simulink model "lin_feedback_EMPTY (1)"  (R2021b)
settings: Solver=ode1  StartTime=0.0  StopTime=tmax  FixedStep=Ts  RelTol=1e-3  EnableMultiTasking=on
values from neighbouring files (symbols this model uses):
  Kd = 0.5    [nlc_setup_solucion (1).m]    (also in nlc_setup_solucion.m = 2)
  Ki = 0    [nlc_setup_solucion (1).m]    (also in nlc_setup_solucion.m = 1)
  Kp = 1    [nlc_setup_solucion (1).m]    (also in nlc_setup_solucion.m = 2.5)
  spd_b = 0    [nlc_setup_solucion (1).m]
  spd_Kaw = spd_aw*spd_Ki/spd_Kp    (= 13.2992871582)    [nlc_setup_solucion (1).m]
  spd_Ki = wn_w^2/b_w    (= 2.87757197383)    [nlc_setup_solucion (1).m]
  spd_Kp = (2*zeta_w*wn_w - a_w)/b_w    (= 0.216370391856)    [nlc_setup_solucion (1).m]
  tau_lpf = 0    [nlc_setup_solucion (1).m]
  Ts = 0.002    [nlc_setup_solucion (1).m]    (also in nlc_setup_solucion.m)
  w_max = 380    [nlc_setup_solucion (1).m]
  w_tau = 20    [nlc_setup_solucion (1).m]    (also in nlc_setup_solucion.m = 5)
undefined symbols (not defined in the file or in its folder): DiscIntNeverNeededParam, HIL, qc_get_step_size
libraries: quarc_library x6
settings Model: SimulationMode=external  ExtModeTrigDuration=20000  Creator=MLevis  LastModifiedBy=Professorat
settings SolverCC: AlgebraicLoopSolver=TrustRegion  PositivePriorityOrder=on  AutoInsertRateTranBlk=on
settings DataIOCC: LimitDataPoints=on  SaveFormat=StructureWithTime  ReturnWorkspaceOutputs=off
settings DebuggingCC: SolverPrmCheckMsg=warning  SFUnexpectedBacktrackingDiag=warning  SFNoUnconditionalDefaultTransitionDiag=warning  SFExecutionAtInitializationDiag=none  SFMachineParentedDataDiag=warning  ArithmeticOperatorsInVariantConditions=warning
settings ModelReferenceCC: PropagateSignalLabelsOutOfModel=off
settings SFSimCC: SimUseLocalCustomCode=off  CustomCodeUndefinedFunction=UseInterfaceOnly
settings RTWCC: Description=QUARC Win64 Target Using Toolchain  SystemTargetFile=quarc_win64.tlc  TemplateMakefile=quarc_default_tmf  RTWUseLocalCustomCode=off  Toolchain=QUARC win64 | nmake (64-bit Windows)  BuildConfiguration=Faster Runs
settings CodeAppCC: StateflowObjectComments=on
settings STFCustomTargetCC: ConcurrentExecutionCompliant=on  UseToolchainInfoCompliant=on  SystemTargetFile=quarc_win64.tlc
settings GRTTargetCC: TargetLangStandard=C89/C90 (ANSI)  ParMdlRefBuildCompliant=off  CompOptLevelCompliant=off  CombineOutputUpdateFcns=off  MatFileLogging=off  CPPClassGenCompliant=off  GRTInterface=on  ExtMode=on  ExtModeMexFile=quarc_comm
settings ConfigComp: CovMetricSettings=dw  CovSaveCumulativeToWorkspaceVar=on  CovSaveSingleToWorkspaceVar=on  CovExternalEMLEnable=off  CovSFcnEnable=off

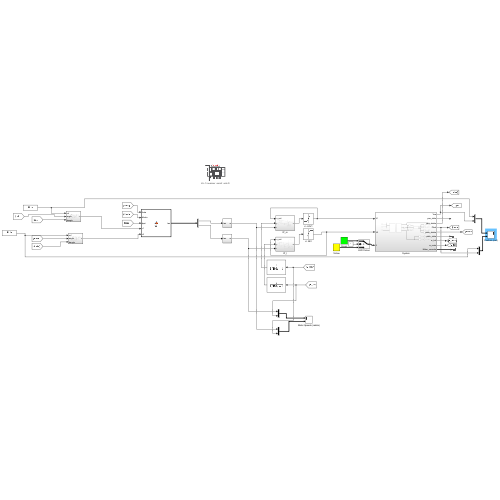
[thumbnail: Simulink's stored preview of the top-level diagram]
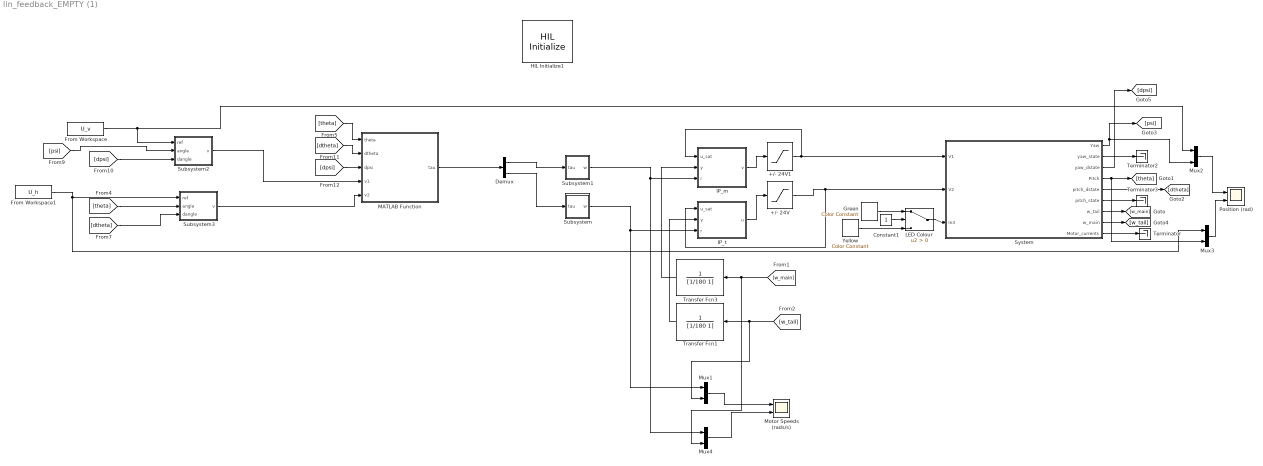
== system lin_feedback_EMPTY (1) ==
  +/- 24V : Saturate  UpperLimit=24  LowerLimit=-24
  +/- 24V1 : Saturate  UpperLimit=24  LowerLimit=-24
  Constant1 : Constant
  Demux : Demux  Outputs=2
  From Workspace : FromWorkspace  VariableName=U_v  Interpolate=off  OutputAfterFinalValue=Setting to zero
  From Workspace1 : FromWorkspace  VariableName=U_h  Interpolate=off  OutputAfterFinalValue=Setting to zero
  Green : quarc_library/Sources/Signals/Color Constant  color=[0 1 0]
      settings: SourceProductName=QUARC Targets
  HIL Initialize1 : quarc_library/Data Acquisition/Generic/Configuration/HIL Initialize  Priority=-99  object_name=HIL-1  board_type=quanser_aero2_usb  board_number=0  board_options=""  exclusive=off  active=off  hardware_clocks=[0]  clock_modes=[]  initial_clock_frequencies=[]  set_clock_params_at_start=off  set_clock_params_at_switch_in=off  set_clock_frequencies_at_start=off  set_clock_frequencies_at_switch_in=off  analog_input_channels=[0:1]  analog_input_configurations=[]  analog_input_maximums=3  analog_input_minimums=-3  set_analog_input_params_at_start=off  set_analog_input_params_at_switch_in=off  analog_output_channels=[0:1]  analog_output_maximums=24  analog_output_minimums=-24  initial_analog_outputs=[0]  final_analog_outputs=[0]  watchdog_analog_outputs=[0]  set_analog_output_params_at_start=off  set_analog_output_params_at_switch_in=off  set_analog_outputs_at_start=on  set_analog_outputs_at_switch_in=off  set_analog_outputs_at_terminate=on  set_analog_outputs_at_switch_out=off  set_analog_outputs_on_watchdog=on  digital_input_channels=[]  digital_output_channels=[0:1]  digital_output_configuration=[]  initial_digital_outputs=[1]  final_digital_outputs=[0]  watchdog_digital_outputs=[0]  set_digital_output_params_at_start=off  set_digital_output_params_at_switch_in=off  set_digital_outputs_at_start=on  set_digital_outputs_at_switch_in=off  set_digital_outputs_at_terminate=on  set_digital_outputs_at_switch_out=off  set_digital_outputs_on_watchdog=on  encoder_channels=[0:3]  quadrature=[4]  encoder_filter_frequency=[]  initial_encoder_counts=[0]  set_encoder_params_at_start=off  set_encoder_params_at_switch_in=off  set_encoder_counts_at_start=on  set_encoder_counts_at_switch_in=off  pwm_channels=[]  pwm_modes=[]  pwm_frequency=[]  pwm_configuration=[]  pwm_alignment=[]  pwm_polarity=[]  pwm_leading_deadband=[]  pwm_trailing_deadband=[]  initial_pwm_outputs=[]  final_pwm_outputs=[]  watchdog_pwm_outputs=[]  set_pwm_params_at_start=off  set_pwm_params_at_switch_in=off  set_pwm_outputs_at_start=off  set_pwm_outputs_at_switch_in=off  set_pwm_outputs_at_terminate=off  set_pwm_outputs_at_switch_out=off  set_pwm_outputs_on_watchdog=off  other_output_channels=[11000:11002]  initial_other_outputs=[0 1 0]  final_other_outputs=[1 0 0]  watchdog_other_outputs=[0 0 1]  set_other_outputs_at_start=on  set_other_outputs_at_switch_in=off  set_other_outputs_at_terminate=on  set_other_outputs_at_switch_out=off  set_other_outputs_on_watchdog=on
  IP_m : Subsystem
  IP_t : Subsystem
  LED Colour : Switch  Criteria=u2 > Threshold
  MATLAB Function : MATLAB Function  TreatAsAtomicUnit=on
  Motor Speeds (rads/s) : Scope  NumInputPorts=2
  Mux{1..4} (4 alike) : Mux  Inputs=2
  Position (rad) : Scope  NumInputPorts=2
  Subsystem : Subsystem
  Subsystem1 : Subsystem
  Subsystem2 : Subsystem
  Subsystem3 : Subsystem
  System : Subsystem
  Terminator : Terminator
  Terminator2 : Terminator
  Terminator3 : Terminator
  Transfer Fcn1 : TransferFcn  Denominator=[1/180 1]
  Transfer Fcn3 : TransferFcn  Denominator=[1/180 1]
  Yellow : quarc_library/Sources/Signals/Color Constant  color=[1 1 0]
      settings: SourceProductName=QUARC Targets
  wires:
  Green/1 -> LED Colour/1
  Yellow/1 -> LED Colour/3
  Constant1/1 -> LED Colour/2
  +/- 24V/1 -> IP_t/1(u_sat), System/2(V2)
  +/- 24V1/1 -> IP_m/1(u_sat), System/1(V1)
  IP_t/1(u) -> +/- 24V/1
  Mux1/1 -> Motor Speeds (rads/s)/1
  Mux4/1 -> Motor Speeds (rads/s)/2
  LED Colour/1 -> System/3(In3)
  System/7(w_tail) -> [w_main]
  System/8(w_main) -> [w_tail]
  System/9(Motor_currents) -> Terminator/1
  System/1(Yaw) -> [psi], Mux2/2
  System/2(yaw_state) -> Terminator2/1
  System/6(pitch_state) -> Terminator3/1
  [w_main] -> Mux4/2, Transfer Fcn3/1
  [w_tail] -> Mux1/2, Transfer Fcn1/1
  Subsystem1/1(w) -> Mux4/1, IP_m/3(r)
  Subsystem/1(w) -> Mux1/1, IP_t/3(r)
  Transfer Fcn1/1 -> IP_t/2(y)
  System/4(Pitch) -> Mux3/2, [theta]
  System/5(pitch_dstate) -> [dtheta]
  System/3(yaw_dstate) -> [dpsi]
  [theta] -> Subsystem3/2(angle)
  [dtheta] -> Subsystem3/3(dangle)
  [psi] -> Subsystem2/2(angle)
  [dpsi] -> Subsystem2/3(dangle)
  From Workspace1/1 -> Mux3/1, Subsystem3/1(ref)
  From Workspace/1 -> Subsystem2/1(ref), Mux2/1
  Mux2/1 -> Position (rad)/1
  Mux3/1 -> Position (rad)/2
  Demux/1 -> Subsystem1/1(tau)
  [dtheta] -> MATLAB Function/2(dtheta)
  Subsystem3/1(v) -> MATLAB Function/5(v2)
  Demux/2 -> Subsystem/1(tau)
  [theta] -> MATLAB Function/1(theta)
  [dpsi] -> MATLAB Function/3(dpsi)
  Subsystem2/1(v) -> MATLAB Function/4(v1)
  MATLAB Function/1(tau) -> Demux/1
  IP_m/1(v) -> +/- 24V1/1
  Transfer Fcn3/1 -> IP_m/2(y)

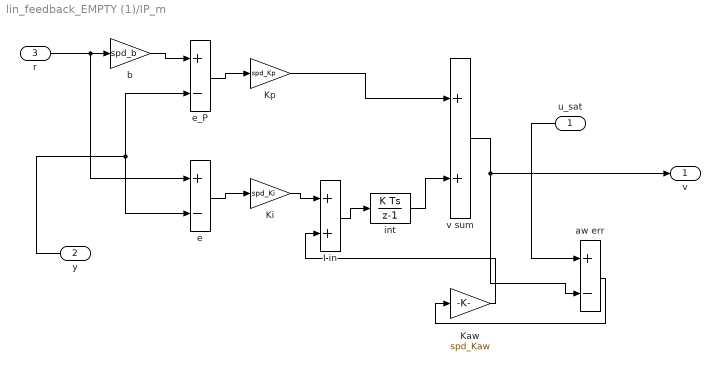
== system lin_feedback_EMPTY (1)/IP_m ==
  u_sat : Inport
  y : Inport  Port=2
  r : Inport  Port=3
  I in : Sum
  Kaw : Gain  Gain=spd_Kaw
  Ki : Gain  Gain=spd_Ki
  Kp : Gain  Gain=spd_Kp
  aw err : Sum  Inputs=+-
  b : Gain  Gain=spd_b
  e : Sum  Inputs=+-
  e_P : Sum  Inputs=+-
  int : DiscreteIntegrator  SampleTime=Ts  ICPrevOutput=DiscIntNeverNeededParam  ICPrevScaledInput=DiscIntNeverNeededParam
  v sum : Sum
  v : Outport
  wires:
  e_P/1 -> Kp/1
  r/1 -> b/1, e/1
  v sum/1 -> aw err/2, v/1
  Kaw/1 -> I in/2
  Kp/1 -> v sum/1
  int/1 -> v sum/2
  aw err/1 -> Kaw/1
  y/1 -> e_P/2, e/2
  I in/1 -> int/1
  e/1 -> Ki/1
  b/1 -> e_P/1
  Ki/1 -> I in/1
  u_sat/1 -> aw err/1

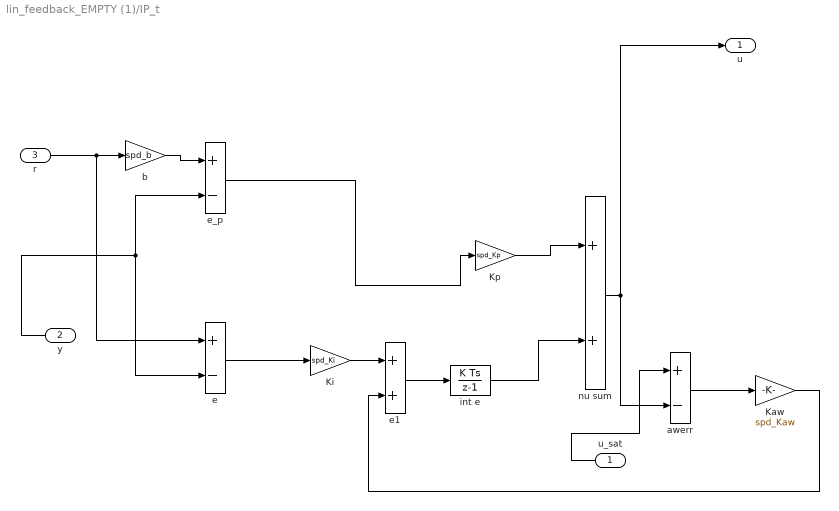
== system lin_feedback_EMPTY (1)/IP_t ==
  u_sat : Inport
  y : Inport  Port=2
  r : Inport  Port=3
  Kaw : Gain  Gain=spd_Kaw
  Ki : Gain  Gain=spd_Ki
  Kp : Gain  Gain=spd_Kp
  awerr : Sum  Inputs=+-
  b : Gain  Gain=spd_b
  e : Sum  Inputs=+-
  e1 : Sum
  e_p : Sum  Inputs=+-
  int e : DiscreteIntegrator  SampleTime=Ts  ICPrevOutput=DiscIntNeverNeededParam  ICPrevScaledInput=DiscIntNeverNeededParam
  nu sum : Sum
  u : Outport
  wires:
  r/1 -> e/1, b/1
  y/1 -> e_p/2, e/2
  b/1 -> e_p/1
  e_p/1 -> Kp/1
  e/1 -> Ki/1
  Ki/1 -> e1/1
  e1/1 -> int e/1
  Kp/1 -> nu sum/1
  int e/1 -> nu sum/2
  nu sum/1 -> u/1, awerr/2
  u_sat/1 -> awerr/1
  awerr/1 -> Kaw/1
  Kaw/1 -> e1/2

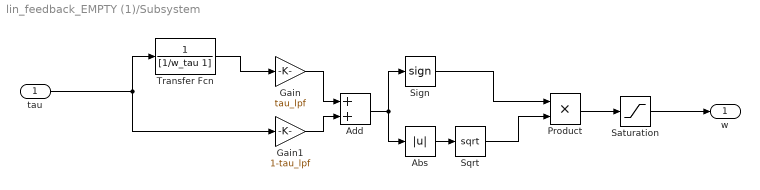
== system lin_feedback_EMPTY (1)/Subsystem ==
  tau : Inport
  Abs : Abs
  Add : Sum
  Gain : Gain  Gain=tau_lpf
  Gain1 : Gain  Gain=1-tau_lpf
  Product : Product
  Saturation : Saturate  UpperLimit=w_max  LowerLimit=-w_max
  Sign : Signum
  Sqrt : Sqrt  SaturateOnIntegerOverflow=on
  Transfer Fcn : TransferFcn  Denominator=[1/w_tau 1]
  w : Outport
  wires:
  Transfer Fcn/1 -> Gain/1
  tau/1 -> Transfer Fcn/1, Gain1/1
  Product/1 -> Saturation/1
  Sign/1 -> Product/1
  Add/1 -> Sign/1, Abs/1
  Sqrt/1 -> Product/2
  Abs/1 -> Sqrt/1
  Gain1/1 -> Add/2
  Gain/1 -> Add/1
  Saturation/1 -> w/1

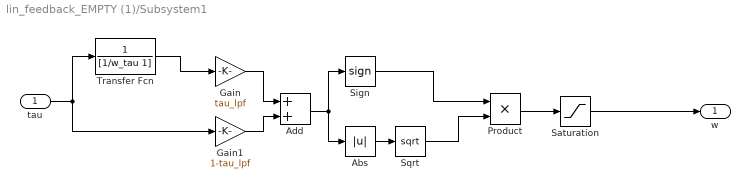
== system lin_feedback_EMPTY (1)/Subsystem1 ==
  tau : Inport
  Abs : Abs
  Add : Sum
  Gain : Gain  Gain=tau_lpf
  Gain1 : Gain  Gain=1-tau_lpf
  Product : Product
  Saturation : Saturate  UpperLimit=w_max  LowerLimit=-w_max
  Sign : Signum
  Sqrt : Sqrt  SaturateOnIntegerOverflow=on
  Transfer Fcn : TransferFcn  Denominator=[1/w_tau 1]
  w : Outport
  wires:
  tau/1 -> Transfer Fcn/1, Gain1/1
  Transfer Fcn/1 -> Gain/1
  Gain1/1 -> Add/2
  Gain/1 -> Add/1
  Add/1 -> Sign/1, Abs/1
  Abs/1 -> Sqrt/1
  Sign/1 -> Product/1
  Sqrt/1 -> Product/2
  Product/1 -> Saturation/1
  Saturation/1 -> w/1

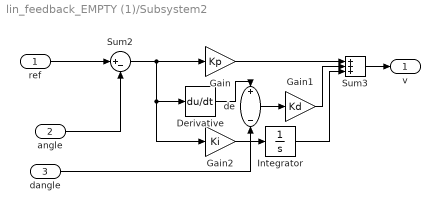
== system lin_feedback_EMPTY (1)/Subsystem2 ==
  ref : Inport
  angle : Inport  Port=2
  dangle : Inport  Port=3
  Derivative : Derivative
  Gain : Gain  Gain=Kp
  Gain1 : Gain  Gain=Kd
  Gain2 : Gain  Gain=Ki
  Integrator : Integrator
  Sum2 : Sum  Inputs=|+-
  Sum3 : Sum  Inputs=+++
  de : Sum  Description=Kd term: d(ref)/dt - measured rate (no derivative of the quantized error)  Inputs=+-
  v : Outport
  wires:
  Sum2/1 -> Gain/1, Derivative/1, Gain2/1
  Gain/1 -> Sum3/1
  ref/1 -> Sum2/1
  Gain1/1 -> Sum3/2
  angle/1 -> Sum2/2
  Sum3/1 -> v/1
  Gain2/1 -> Integrator/1
  Integrator/1 -> Sum3/3
  Derivative/1 -> de/1
  de/1 -> Gain1/1
  dangle/1 -> de/2

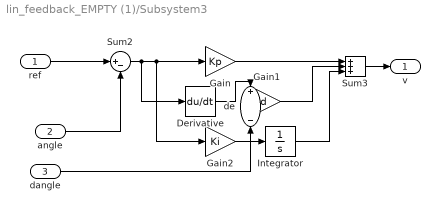
== system lin_feedback_EMPTY (1)/Subsystem3 ==
  ref : Inport
  angle : Inport  Port=2
  dangle : Inport  Port=3
  Derivative : Derivative
  Gain : Gain  Gain=Kp
  Gain1 : Gain  Gain=Kd
  Gain2 : Gain  Gain=Ki
  Integrator : Integrator
  Sum2 : Sum  Inputs=|+-
  Sum3 : Sum  Inputs=+++
  de : Sum  Description=Kd term: d(ref)/dt - measured rate (no derivative of the quantized error)  Inputs=+-
  v : Outport
  wires:
  Sum2/1 -> Derivative/1, Gain/1, Gain2/1
  Gain/1 -> Sum3/1
  ref/1 -> Sum2/1
  Gain1/1 -> Sum3/2
  angle/1 -> Sum2/2
  Sum3/1 -> v/1
  Gain2/1 -> Integrator/1
  Integrator/1 -> Sum3/3
  Derivative/1 -> de/1
  de/1 -> Gain1/1
  dangle/1 -> de/2

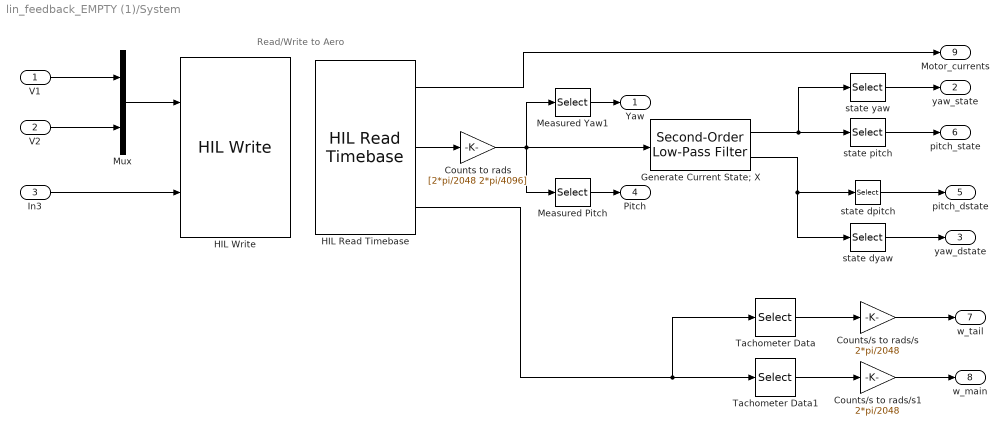
== system lin_feedback_EMPTY (1)/System ==
  note: Read/Write to Aero
  V1 : Inport
  V2 : Inport  Port=2
  In3 : Inport  Port=3
  Counts to rads : Gain  Gain=[2*pi/2048 2*pi/4096]
  Counts/s to rads/s : Gain  Gain=2*pi/2048
  Counts/s to rads/s1 : Gain  Gain=2*pi/2048
  Generate Current State; X : quarc_library/Continuous/Second-Order Low-Pass Filter  params_source=Internal (dialog parameters)  input_width=10  input_zeta=0.8  input_init=0
  HIL Read Timebase : quarc_library/Data Acquisition/Generic/Timebases/HIL Read Timebase  object_name=HIL-1  clock=0  analog_channels=[0:1]  encoder_channels=[2:3]  digital_channels=[]  other_channels=[4000 4002 14000 14001]  active=on  vector_output=on  data_type_mode=Inherit via back propagation  encoder_data_type=double  digital_data_type=boolean  overflow_mode=Error on overflow  samples_in_buffer=max(ceil(1/qc_get_step_size), 1)
  HIL Write : quarc_library/Data Acquisition/Generic/Immediate I//O/HIL Write  object_name=HIL-1  analog_channels=[0:1]  pwm_channels=[]  digital_channels=[]  other_channels=[11000:11002]  sample_time=-1  active=off  vector_input=on
  Measured Pitch : Selector  InputPortWidth=2  IndexOptions=Index vector (dialog)  Indices=[1]  OutputSizes=1
  Measured Yaw1 : Selector  InputPortWidth=2  IndexOptions=Index vector (dialog)  Indices=[2]  OutputSizes=1
  Mux : Mux  Inputs=2
  Tachometer Data : Selector  InputPortWidth=4  IndexOptions=Index vector (dialog)  Indices=[3]  OutputSizes=1
  Tachometer Data1 : Selector  InputPortWidth=4  IndexOptions=Index vector (dialog)  Indices=[4]  OutputSizes=1
  state dpitch : Selector  InputPortWidth=2  IndexOptions=Index vector (dialog)  Indices=[1]  OutputSizes=1
  state dyaw : Selector  InputPortWidth=2  IndexOptions=Index vector (dialog)  Indices=[2]  OutputSizes=1
  state pitch : Selector  InputPortWidth=2  IndexOptions=Index vector (dialog)  Indices=[1]  OutputSizes=1
  state yaw : Selector  InputPortWidth=2  IndexOptions=Index vector (dialog)  Indices=[2]  OutputSizes=1
  Yaw : Outport
  yaw_state : Outport  Port=2
  yaw_dstate : Outport  Port=3
  Pitch : Outport  Port=4
  pitch_dstate : Outport  Port=5
  pitch_state : Outport  Port=6
  w_tail : Outport  Port=7
  w_main : Outport  Port=8
  Motor_currents : Outport  Port=9
  wires:
  state dpitch/1 -> pitch_dstate/1
  Generate Current State; X/1 -> state yaw/1, state pitch/1
  V1/1 -> Mux/1
  Counts to rads/1 -> Measured Pitch/1, Generate Current State; X/1, Measured Yaw1/1
  Mux/1 -> HIL Write/1
  HIL Read Timebase/2 -> Counts to rads/1
  In3/1 -> HIL Write/2
  Generate Current State; X/2 -> state dyaw/1, state dpitch/1
  HIL Read Timebase/1 -> Motor_currents/1
  state yaw/1 -> yaw_state/1
  V2/1 -> Mux/2
  Measured Pitch/1 -> Pitch/1
  state pitch/1 -> pitch_state/1
  state dyaw/1 -> yaw_dstate/1
  Measured Yaw1/1 -> Yaw/1
  Counts/s to rads/s/1 -> w_tail/1
  Tachometer Data1/1 -> Counts/s to rads/s1/1
  Counts/s to rads/s1/1 -> w_main/1
  HIL Read Timebase/3 -> Tachometer Data/1, Tachometer Data1/1
  Tachometer Data/1 -> Counts/s to rads/s/1

== matlab function lin_feedback_EMPTY (1)/MATLAB Function ==
  data: theta input; tau output; dtheta input; dpsi input; v1 input; v2 input
function tau = fcn(theta,dtheta,dpsi,v1,v2)

Jph = 0.6407;
jph = 0.01;
Jth = 0.7164;
Dph = 0;          % B_q = 0 (aero2_model.pdf)
Dth = 0;
Cor = Jph - jph;

L = 0.167;
G = 0.0254;
kF=2.5526e-5;
kT=4.2487e-6;


%% FEEDBACK LINEARISATION (same law as block "Feedback linearization" of the simulation)
%   Mq(q) ddq + cq(q,dq) + Bq dq + gq(q) = Gamma(theta) tau ,   tau = [wm|wm| ; wt|wt|]
%   tau_d = Gamma(theta)^-1 ( Mq(q) nu + cq + Bq dq + gq )   ==>   ddq = nu
%   The signed square root  w_d = sign(tau_d) sqrt(|tau_d|)  is done afterwards
%   in the "tau -> w" subsystems (Subsystem1 = main, Subsystem = tail).
%   Valid while cos(theta) ~= 0  (|theta| < pi/2).
nu = [v1; v2];                       % outputs of the position controllers [yaw; pitch]
c  = cos(theta);  s = sin(theta);
Mq = [Jph*c^2 + jph*s^2, 0; 0, Jth];
cq = [-Cor*sin(2*theta)*dtheta*dpsi; 0.5*Cor*sin(2*theta)*dpsi^2];
Bq = [Dph*dpsi; Dth*dtheta];
gq = [0; G*s];
cg = c;                              % guard against the singularity theta = +-pi/2
if abs(cg) < 0.1
    cg = 0.1*sign(cg + (cg == 0));
end
Gam = [-cg*kT, cg*L*kF; L*kF, kT];   % Gamma(theta) = [c 0; 0 1]*[-kT L*kF; L*kF kT]
tau = Gam \ (Mq*nu + cq + Bq + gq);  % tau(1) -> main rotor, tau(2) -> tail rotors
